simulink model "sensor_real_posicion_LU"  (R2026b)
settings: Solver=VariableStepAuto
values from neighbouring files (symbols this model uses):
  wn_E = 2000    [coeficientes.m]
  zeta_E = 1    [coeficientes.m]
settings Model: Creator=lamun  LastModifiedBy=lamun

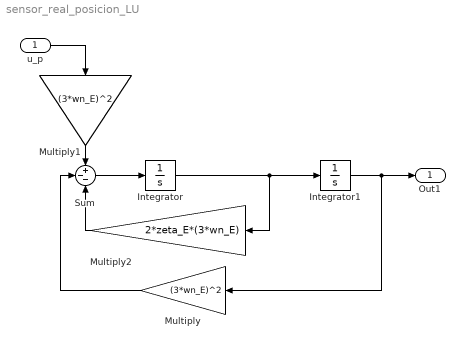
== system sensor_real_posicion_LU ==
  u_p : Inport
  Integrator : Integrator
  Integrator1 : Integrator
  Multiply : Gain  Gain=(3*wn_E)^2
  Multiply1 : Gain  Gain=(3*wn_E)^2
  Multiply2 : Gain  Gain=2*zeta_E*(3*wn_E)
  Sum : Sum  Inputs=+--
  Out1 : Outport
  wires:
  Multiply1/1 -> Sum/1
  u_p/1 -> Multiply1/1
  Sum/1 -> Integrator/1
  Integrator/1 -> Multiply2/1, Integrator1/1
  Multiply2/1 -> Sum/3
  Multiply/1 -> Sum/2
  Integrator1/1 -> Out1/1, Multiply/1
